simulink model "ProjectModel"  (R2024a)
settings: Solver=VariableStepAuto  StartTime=0.0  StopTime=5  RelTol=1e-3
model workspace (MAT data in the model file):
  L = 0.5
  M = 0.5
  Q = 21
  Ts = 0.01
  b = 0.1
  g = 9.8
  l = 0.5
  m = 0.2
  theta0 = 2.82743338823
settings Model: Creator=sturton  LastModifiedBy=DELL
settings ConfigComp: CovMetricSettings=de

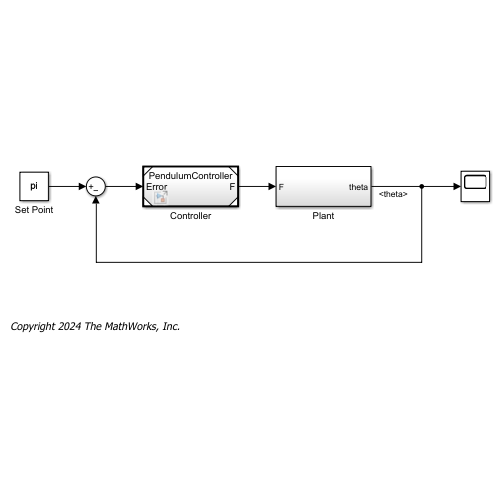
[thumbnail: Simulink's stored preview of the top-level diagram]
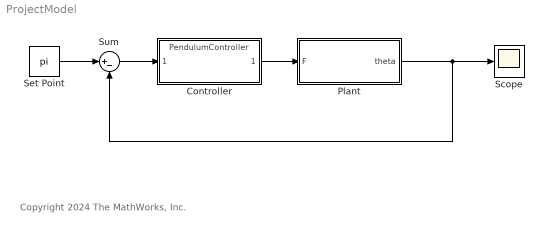
== system ProjectModel ==
  note: Copyright 2024 The MathWorks, Inc.
  Controller : ModelReference  ModelNameDialog=PendulumController.slx  SimulationMode=Normal  ModelReferenceVersion=1.1
  Plant : Subsystem
  Scope : Scope
  Set Point : Constant  Value=pi
  Sum : Sum  Inputs=|+-
  wires:
  Plant/1(theta) -> Scope/1, Sum/2
  Set Point/1 -> Sum/1
  Sum/1 -> Controller/1
  Controller/1 -> Plant/1(F)

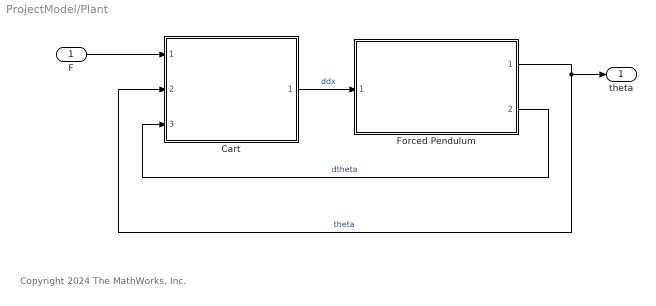
== system ProjectModel/Plant ==
  note: Copyright 2024 The MathWorks, Inc.
  F : Inport
  Cart : Subsystem  ReferencedSubsystem=CartBase
  Forced Pendulum : Subsystem  ReferencedSubsystem=InvertedPendulum
  theta : Outport
  wires:
  F/1 -> Cart/1
  Cart/1 -> Forced Pendulum/1  "ddx"
  Forced Pendulum/1 -> Cart/2, theta/1  "theta"
  Forced Pendulum/2 -> Cart/3  "dtheta"
